simulink model "ADCSSimulator"  (R2024a)
settings: Solver=ode4  StartTime=0.0  StopTime=600  FixedStep=0.01  MaxStep=0.1  RelTol=1e-3  AbsTol=1e-3
values from neighbouring files (symbols this model uses):
  ActuatorAllocationMatrix = ActuatorPhysicalMatrix' * inv(ActuatorPhysicalMatrix * ActuatorPhysicalMatrix')    [set_Init.m]
  ActuatorPhysicalMatrix = [1, 0, 0, 0 ... (first row only)    [set_Init.m]
  albedo_irradiance = 300    [set_Init.m]
  b = 0    [set_Init.m]
  Cd = 2.2    [set_Init.m]
  h_bias = [0; 0; 0]    [set_Init.m]
  J = 4.0e-3 / 628    (= 6.36942675159e-06)    [set_Init.m]
  k_Bdot = ((4 * pi * 0.5236 * 0.0055) / (5677.2 * (4.5e-5)^2))    (= 3147.8423197)    [set_Init.m]
  K_E = K_T    (= 0.0022)    [set_Init.m]
  K_T = 0.0022    [set_Init.m]
  P0 = blkdiag(P0_att, P0_bias)    [set_Init.m]
  P0_att = eye(3) * initial_variance_rad2    [set_Init.m]
  PowerVoltageBus_01 = 3.3    [set_Init.m]
  PowerVoltageBus_02 = 3.3    [set_Init.m]
  PowerVoltageBus_03 = 3.3    [set_Init.m]
  PowerVoltageBus_04 = 3.3    [set_Init.m]
  PowerVoltageBus_05 = 3.3    [set_Init.m]
  PowerVoltageBus_06 = 3.3    [set_Init.m]
  PowerVoltageBus_07 = 3.3    [set_Init.m]
  PowerVoltageBus_08 = 3.3    [set_Init.m]
  PowerVoltageBus_09 = 3.3    [set_Init.m]
  PowerVoltageBus_10 = 3.3    [set_Init.m]
  PowerVoltageBus_11 = 3.3    [set_Init.m]
  PowerVoltageBus_12 = 0.0    (= 0)    [set_Init.m]
  PowerVoltageBus_13 = 0.0    (= 0)    [set_Init.m]
  PowerVoltageBus_14 = 0.0    (= 0)    [set_Init.m]
  PowerVoltageBus_15 = 0.0    (= 0)    [set_Init.m]
  R = 2.0    (= 2)    [set_Init.m]
  ressidual_m = [3e-4; -2e-4; 1e-4]    [set_Init.m]
  solar_irradiance = 1361    [set_Init.m]
  surface_areas = [A_xy, A_yz, A_xz, A_xy, A_yz, A_xz]    [set_Init.m]
  surface_normals_body = [eye(3) -eye(3)]    [set_Init.m]
  surface_positions_body = [       hx,   0,   0 ... (first row only)    [set_Init.m]
  surface_reflectivities = [0.9 0.8 0.9 0.9 0.9 0.9]    [set_Init.m]
  Switch_01 = 1    [set_Init.m]
  Switch_02 = 1    [set_Init.m]
  Switch_03 = 1    [set_Init.m]
  Switch_04 = 1    [set_Init.m]
  Switch_05 = 1    [set_Init.m]
  Switch_06 = 1    [set_Init.m]
  Switch_07 = 1    [set_Init.m]
  Switch_08 = 1    [set_Init.m]
  Switch_09 = 1    [set_Init.m]
  Switch_10 = 1    [set_Init.m]
  Switch_11 = 1    [set_Init.m]
  Switch_12 = 0    [set_Init.m]
  Switch_13 = 0    [set_Init.m]
  Switch_14 = 0    [set_Init.m]
  Switch_15 = 0    [set_Init.m]
  visSampleTime = 0.1    [set_Init.m]
undefined symbols (not defined in the file or in its folder): attitude, Controller, epoch, IAU, juliandate, Kd, km, Kp, m, rad, s, satellite, SGP4_parameters, simulator, UKF_parameters, WMM2020
libraries: sharedtransform x27, aerolibutil x22, aerolibconvert2 x18, simulink_extras x16, matrix_library x6, aerolibtransform2 x4, vrlib x2, aerolibgravity2 x2, aerolibobsolete x1, aerolibattitudesys x1, simulink x1
(part 1 of 8)
settings Model: Creator=dani  LastModifiedBy=dani

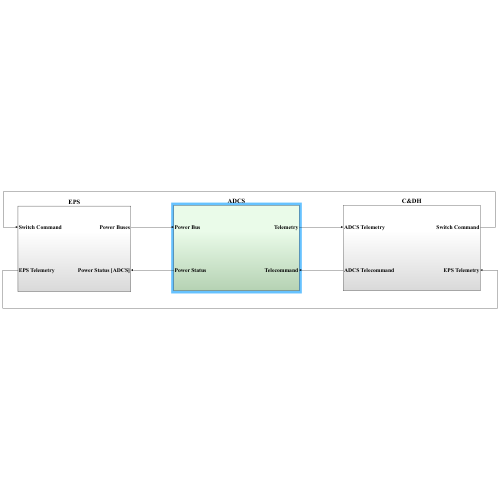
[thumbnail: Simulink's stored preview of the top-level diagram]
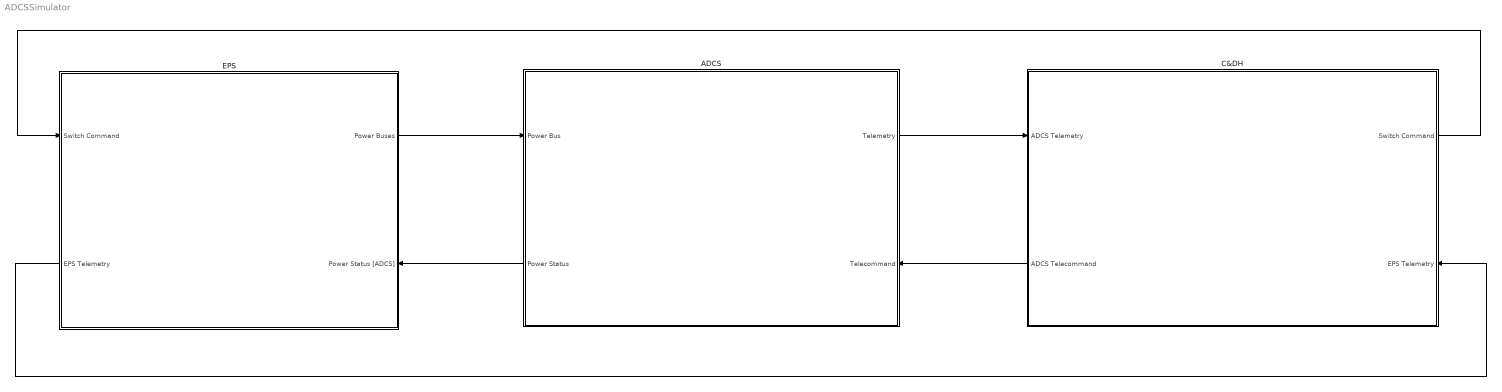
== system ADCSSimulator ==
  ADCS : Subsystem
      settings: PortSchema="{\"entries\":[{\"content\":{\"sides\":[{\"content\":{\"connectorIds\":[\"In1\",\"Out2\"]},\"type\":\"ConnectorPlacement.EquallySpacedRectSide\",\"uuid\":\"aa3848c2-740f-4ead-a432-f3c79fc9daf0\"},{\"content\":{\"connectorIds\":[\"Out1\",\"In2\"],\"side\":\"RIGHT\"},\"type\":\"ConnectorPlacement.EquallySpacedRectSide\",\"uuid\":\"c96c275d-03b5-4d03-9fcd-7be32dac6d00\"},{\"content\":{\"side\":\"TOP\"},\"type\":\"ConnectorPlacement.EquallySpacedRectSide\",\"uuid\":\"31331525-31c2-42c0-b454-d98af43a0c1b\"},{\"content\":{\"side\":\"BOTTOM\"},\"type\":\"ConnectorPlacement.EquallySpacedRectSide\",\"uuid\":\"eb70cc62-5643-48b5-a59b-44e32afdbd5b\"}]},\"type\":\"ConnectorPlacement.EquallySpacedConnector\",\"uuid\":\"a031f488-e476-44b2-bfa5-ca27c87ecf65\"}],\"packageUris\":[\"http://schema.mathworks.com/mf0/Connector/R2020b\"],\"version\":\"1.0\"}"
  C&DH : Subsystem
      settings: PortSchema="{\"entries\":[{\"content\":{\"sides\":[{\"content\":{\"connectorIds\":[\"In1\",\"Out2\"]},\"type\":\"ConnectorPlacement.EquallySpacedRectSide\",\"uuid\":\"3ad3e378-21eb-4eff-b41a-c92f181c1ecc\"},{\"content\":{\"connectorIds\":[\"Out1\",\"In2\"],\"side\":\"RIGHT\"},\"type\":\"ConnectorPlacement.EquallySpacedRectSide\",\"uuid\":\"0538179f-4ab0-45db-a75e-d38723b4a5a1\"},{\"content\":{\"side\":\"TOP\"},\"type\":\"ConnectorPlacement.EquallySpacedRectSide\",\"uuid\":\"084a5a74-d737-4e15-943a-c0ca9c781568\"},{\"content\":{\"side\":\"BOTTOM\"},\"type\":\"ConnectorPlacement.EquallySpacedRectSide\",\"uuid\":\"08c1cc82-b359-4a4d-a3dd-2424cb8433d7\"}]},\"type\":\"ConnectorPlacement.EquallySpacedConnector\",\"uuid\":\"d1795a99-1dc8-4811-af35-3434a23822bd\"}],\"packageUris\":[\"http://schema.mathworks.com/mf0/Connector/R2020b\"],\"version\":\"1.0\"}"
  EPS : Subsystem
      settings: PortSchema="{\"entries\":[{\"content\":{\"sides\":[{\"content\":{\"connectorIds\":[\"In1\",\"Out2\"]},\"type\":\"ConnectorPlacement.EquallySpacedRectSide\",\"uuid\":\"3ad3e378-21eb-4eff-b41a-c92f181c1ecc\"},{\"content\":{\"connectorIds\":[\"Out1\",\"In2\"],\"side\":\"RIGHT\"},\"type\":\"ConnectorPlacement.EquallySpacedRectSide\",\"uuid\":\"0538179f-4ab0-45db-a75e-d38723b4a5a1\"},{\"content\":{\"side\":\"TOP\"},\"type\":\"ConnectorPlacement.EquallySpacedRectSide\",\"uuid\":\"084a5a74-d737-4e15-943a-c0ca9c781568\"},{\"content\":{\"side\":\"BOTTOM\"},\"type\":\"ConnectorPlacement.EquallySpacedRectSide\",\"uuid\":\"08cac11b-dd67-4d0a-9adb-ddefdbada8d1\"}]},\"type\":\"ConnectorPlacement.EquallySpacedConnector\",\"uuid\":\"d1795a99-1dc8-4811-af35-3434a23822bd\"}],\"packageUris\":[\"http://schema.mathworks.com/mf0/Connector/R2020b\"],\"version\":\"1.0\"}"
  wires:
  C&DH/2(ADCS Telecommand) -> ADCS/2(Telecommand)
  ADCS/2(Power Status) -> EPS/2(Power Status [ADCS])
  EPS/1(Power Buses) -> ADCS/1(Power Bus)
  C&DH/1(Switch Command) -> EPS/1(Switch Command)
  ADCS/1(Telemetry) -> C&DH/1(ADCS Telemetry)
  EPS/2(EPS Telemetry) -> C&DH/2(EPS Telemetry)

== system ADCSSimulator/ADCS ==
  note: Temporary Signal
      | (Only for Comparison)
  Power Bus : Inport
  Telecommand : Inport  Port=2
  ADCS Hardware : Subsystem
      settings: PortSchema="{\"entries\":[{\"content\":{\"sides\":[{\"content\":{\"connectorIds\":[\"In1\",\"In2\",\"Out3\"]},\"type\":\"ConnectorPlacement.EquallySpacedRectSide\",\"uuid\":\"766d0d2c-d357-4ba2-aa5f-dc26e66264eb\"},{\"content\":{\"connectorIds\":[\"Out1\",\"Out2\",\"In3\"],\"side\":\"RIGHT\"},\"type\":\"ConnectorPlacement.EquallySpacedRectSide\",\"uuid\":\"3ef54b5b-eb3f-4ad4-b707-91b0a7134d5c\"},{\"content\":{\"side\":\"TOP\"},\"type\":\"ConnectorPlacement.EquallySpacedRectSide\",\"uuid\":\"06ee7821-1a08-4071-958f-cf5282d5f19e\"}]},\"type\":\"ConnectorPlacement.EquallySpacedConnector\",\"uuid\":\"44073966-09cf-4676-b7c4-ea8934a60606\"}],\"packageUris\":[\"http://schema.mathworks.com/mf0/Connector/R2020b\"],\"version\":\"1.0\"}"
  ADCS Software : Subsystem
      settings: PortSchema="{\"entries\":[{\"content\":{\"sides\":[{\"content\":{\"connectorIds\":[\"In1\",\"In2\"]},\"type\":\"ConnectorPlacement.EquallySpacedRectSide\",\"uuid\":\"a2366055-7441-4d66-9a67-a5a05521bed6\"},{\"content\":{\"connectorIds\":[\"Out1\",\"Out2\"],\"side\":\"RIGHT\"},\"type\":\"ConnectorPlacement.EquallySpacedRectSide\",\"uuid\":\"d11468d0-ec53-4005-81d6-c107e48fef08\"},{\"content\":{\"connectorIds\":[\"In3\",\"In4\"],\"side\":\"TOP\"},\"type\":\"ConnectorPlacement.EquallySpacedRectSide\",\"uuid\":\"0424b65d-589c-439a-af82-86bada1149e6\"}]},\"type\":\"ConnectorPlacement.EquallySpacedConnector\",\"uuid\":\"691de30c-3ace-413d-83af-9a4acbe20075\"}],\"packageUris\":[\"http://schema.mathworks.com/mf0/Connector/R2020b\"],\"version\":\"1.0\"}"
  Environment Model : Subsystem
  Telemetry : Outport
  Power Status : Outport  Port=2
  wires:
  Telecommand/1 -> ADCS Software/1(Command)
  Power Bus/1 -> ADCS Hardware/2(Voltage Bus)
  Environment Model/1(Environment) -> ADCS Software/3(Environment), ADCS Hardware/3(True Physical State)
  ADCS Software/1(Actuators Command) -> ADCS Hardware/1(Control Command)
  ADCS Hardware/1(Actuators Command) -> Environment Model/1(Control Torque), ADCS Software/4(Actuators Feedback)
  ADCS Hardware/3(Sensors Data) -> ADCS Software/2(Sensors Data)
  ADCS Software/2(Telemetry) -> Telemetry/1
  ADCS Hardware/2(Power Status) -> Power Status/1

== system ADCSSimulator/C&DH ==
  ADCS Telemetry : Inport
  EPS Telemetry : Inport  Port=2
  Bus Creator : BusCreator  Inputs=15
  Bus Selector : BusSelector  OutputSignals=SOC,Total Instantaneous Power (W),Total Instantaneous Current (A)
  Constant : Constant  Value=Switch_01
  Constant1 : Constant  Value=Switch_02
  Constant10 : Constant  Value=Switch_11
  Constant11 : Constant  Value=Switch_12
  Constant12 : Constant  Value=Switch_13
  Constant13 : Constant  Value=Switch_14
  Constant14 : Constant  Value=Switch_15
  Constant2 : Constant  Value=Switch_03
  Constant3 : Constant  Value=Switch_04
  Constant4 : Constant  Value=Switch_05
  Constant5 : Constant  Value=Switch_06
  Constant6 : Constant  Value=Switch_07
  Constant7 : Constant  Value=Switch_08
  Constant8 : Constant  Value=Switch_09
  Constant9 : Constant  Value=Switch_10
  System Mode (0: OFF) (1: Detumbling) (2: Nadir Pointing) (3: Sun Pointing) : Constant  Value=0
  Terminator : Terminator
  To Workspace : ToWorkspace  VariableName=SOC  SaveFormat=Timeseries  SampleTime=-1
  To Workspace1 : ToWorkspace  VariableName=totoal_p  SaveFormat=Timeseries  SampleTime=-1
  To Workspace2 : ToWorkspace  VariableName=total_I  SaveFormat=Timeseries  SampleTime=-1
  Switch Command : Outport
  ADCS Telecommand : Outport  Port=2
  wires:
  System Mode (0: OFF) (1: Detumbling) (2: Nadir Pointing) (3: Sun Pointing)/1 -> ADCS Telecommand/1
  Constant11/1 -> Bus Creator/12  "Switch 12"
  Constant4/1 -> Bus Creator/5  "Switch 05"
  Constant9/1 -> Bus Creator/10  "Switch 10"
  Constant14/1 -> Bus Creator/15  "Switch 15"
  Constant2/1 -> Bus Creator/3  "Switch 03"
  Constant7/1 -> Bus Creator/8  "Switch 08"
  Constant/1 -> Bus Creator/1  "Switch 01"
  Bus Creator/1 -> Switch Command/1
  Constant12/1 -> Bus Creator/13  "Switch 13"
  Constant3/1 -> Bus Creator/4  "Switch 04"
  Constant1/1 -> Bus Creator/2  "Switch 02"
  Constant5/1 -> Bus Creator/6  "Switch 06"
  Constant6/1 -> Bus Creator/7  "Switch 07"
  Constant13/1 -> Bus Creator/14  "Switch 14"
  Constant10/1 -> Bus Creator/11  "Switch 11"
  Constant8/1 -> Bus Creator/9  "Switch 09"
  ADCS Telemetry/1 -> Terminator/1
  EPS Telemetry/1 -> Bus Selector/1
  Bus Selector/1 -> To Workspace/1  "<SOC>"
  Bus Selector/2 -> To Workspace1/1  "<Total Instantaneous Power (W)>"
  Bus Selector/3 -> To Workspace2/1  "<Total Instantaneous Current (A)>"

== system ADCSSimulator/EPS ==
  Switch Command : Inport
  Power Status [ADCS] : Inport  Port=2
  EPS HouseKeeping : Subsystem
  Power Distribution Unit (PDU) : Subsystem
  Power Buses : Outport
  EPS Telemetry : Outport  Port=2
  wires:
  Switch Command/1 -> [SwitchCommand], Power Distribution Unit (PDU)/1(Switch Bus)
  [SwitchCommand] -> EPS HouseKeeping/1(Switch Status)
  Power Status [ADCS]/1 -> EPS HouseKeeping/2(Power Status)
  EPS HouseKeeping/1(EPS Telemetry) -> EPS Telemetry/1
  Power Distribution Unit (PDU)/1(Voltage Bus) -> Power Buses/1

== system ADCSSimulator/ADCS/ADCS Hardware ==
  Control Command : Inport
  Voltage Bus : Inport  Port=2
  True Physical State : Inport  Port=3
  Actuators : Subsystem
  Bus Creator : BusCreator  Inputs=3
  Bus Selector1 : BusSelector  OutputSignals=MTQs.MTQs Power Status,RWs.RWs Power Status
  Bus Selector2 : BusSelector  OutputSignals=Sensors Power Status
  Bus Selector3 : BusSelector  OutputSignals=|
      | Calendar,Ephemerides.Satellite Ephemeris [ICRF],Satellite Attitude,Eclipse,Magnetic Field (T).MagneticField
      | (T)[Body],Ephemerides.Planetary Ephemeris [ICRF].Sun Ephemeris [ICRF],Transformers
  Bus Selector4 : BusSelector  OutputSignals=MTQs.Dipoles (Am^2),MTQs.MTQs Power Status.Power Consumption [Magnetorquer Z].Current (A),MTQs.MTQs Power Status.Power Consumption [Magnetorquer Y].Current (A),MTQs.MTQs Power Status.Power Consumption [Magnetorquer X].Current (A),RWs.RWs Angular Velocity [Body].RWs Angular Velocity (RPM).RW#1 Motor Angular Velocity (rad/s),RWs.RWs Angular Velocity [Body].RWs Angular Velocity (RPM).RW#2 Motor Angular Velocity (rad/s),RWs.RWs Angular Velocity [Body].RWs Angular Velocity (RPM).RW#3 Motor Angular Velocity (rad/s),RWs.RWs Torque [Body](Nm)
  Constant1 : Constant  Value=satellite.MM.Temperature
  Constant3 : Constant  Value=satellite.Gyro.MeasurementModelDCM
  Constant4 : Constant  Value=satellite.MM.MeasurementModelDCM
  Mux : Mux  Inputs=3
  Mux1 : Mux  Inputs=3
  "Power Bus{2}" : InportShadow  Port=2
  Sensors : Subsystem
  To Workspace : ToWorkspace  VariableName=MTQ_dipoles  SaveFormat=Timeseries  SampleTime=-1
  To Workspace1 : ToWorkspace  VariableName=MTQ_Current  SaveFormat=Timeseries  SampleTime=-1
  To Workspace2 : ToWorkspace  VariableName=RW_angvel  SaveFormat=Timeseries  SampleTime=-1
  To Workspace3 : ToWorkspace  VariableName=RW_Torque  SaveFormat=Timeseries  SampleTime=-1
  Actuators Command : Outport
  Power Status : Outport  Port=2
  Sensors Data : Outport  Port=3
  wires:
  Voltage Bus/1 -> Actuators/2(Input Bus Voltage (V))
  Control Command/1 -> Actuators/1(Control Command)
  Actuators/1(Actuators) -> [Actuators], Actuators Command/1
  [B_Body] -> Actuators/3(Magnetic Field (T))
  Bus Selector2/1 -> Bus Creator/3  "<Sensors Power Status>"
  [Actuators] -> Bus Selector1/1
  [SensorsData] -> Bus Selector2/1
  Bus Selector1/2 -> Bus Creator/2  "<RWs Power Status>"
  Bus Selector1/1 -> Bus Creator/1  "<MTQs Power Status>"
  Bus Creator/1 -> Power Status/1
  Bus Selector3/5 -> [B_Body], Sensors/5(Magnetic Field (T))  "<MagneticField (T)[Body]>"
  Constant4/1 -> Sensors/9(Measurement Model DCM (MM))
  True Physical State/1 -> Bus Selector3/1
  "Power Bus{2}"/1 -> Sensors/11(Input Bus Voltages (V))
  Constant3/1 -> Sensors/10(Measurement Model DCM (Gyro))
  Bus Selector3/3 -> Sensors/3(Satellite Attitude)  "<Satellite Attitude>"
  Bus Selector3/1 -> Sensors/1(Calendar)  "<Calendar>"
  Constant1/1 -> Sensors/8(MM Temperature)
  Sensors/1(Sensrors Out) -> [SensorsData], Sensors Data/1
  Bus Selector3/6 -> Sensors/6(Sun Ephemeris [ICRF])  "<Sun Ephemeris [ICRF]>"
  Bus Selector3/7 -> Sensors/7(Transformers)  "<Transformers>"
  Bus Selector3/2 -> Sensors/2(Satellite Ephemeris)  "<Satellite Ephemeris [ICRF]>"
  Bus Selector3/4 -> Sensors/4(Eclipse)  "<Eclipse>"
  [Actuators] -> Bus Selector4/1
  Bus Selector4/2 -> Mux/1  "<Current (A)>"
  Bus Selector4/1 -> To Workspace/1  "<Dipoles (Am^2)>"
  Bus Selector4/3 -> Mux/2  "<Current (A)>"
  Bus Selector4/4 -> Mux/3  "<Current (A)>"
  Bus Selector4/6 -> Mux1/2  "<RW#2 Motor Angular Velocity (rad/s)>"
  Bus Selector4/5 -> Mux1/1  "<RW#1 Motor Angular Velocity (rad/s)>"
  Bus Selector4/7 -> Mux1/3  "<RW#3 Motor Angular Velocity (rad/s)>"
  Mux/1 -> To Workspace1/1
  Mux1/1 -> To Workspace2/1
  Bus Selector4/8 -> To Workspace3/1  "<RWs Torque [Body](Nm)>"

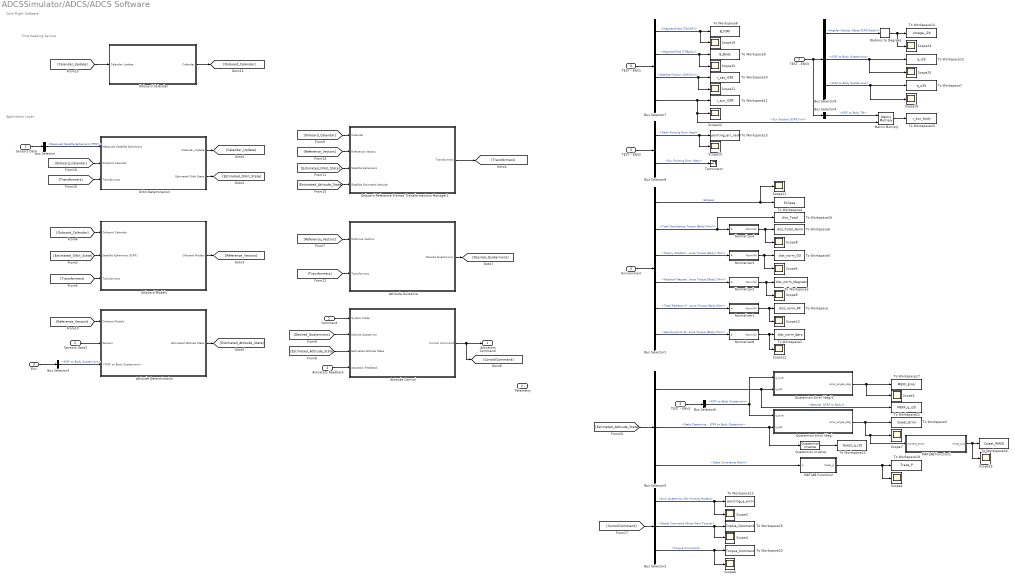
== system ADCSSimulator/ADCS/ADCS Software ==
  note: Time Keeping Service
  note: Core Flight Software
  note: Application Layer
  Command : Inport
  Sensors Data : Inport  Port=2
  Environment : Inport  Port=3
  Actuators Feedback : Inport  Port=4
  Attitude Control : Subsystem
  Attitude Determination : Subsystem
  Attitude Guidance : Subsystem
  Bus Selector : BusSelector  OutputSignals=Measured Satellite Ephemeris [ITRF]
  Bus Selector1 : BusSelector  OutputSignals=Eclipse,Disturbances.Total Disturbance Torque [Body] (Nm),Disturbances.Graciry Gradient Disturbance Torque [Body] (Nm),Disturbances.Residual Magnetic Disturbance Torque [Body] (Nm),Disturbances.Rediation Pressure Torque [Body] (Nm).Total Rediation Pressure Torque [Body](Nm),Disturbances.Aerodynamics Disturbance Torque [Body] (Nm)
  Bus Selector2 : BusSelector  OutputSignals=Error Quaternion [for Pointing Modes],Dipole Command (Given from Torque),Torque Command
  Bus Selector3 : BusSelector  OutputSignals=Transformers.Quaternions.ICRF to Body Quaternions
  Bus Selector4 : BusSelector  OutputSignals=Transformers.Transfer Matrices.ICRF to Body TM
  Bus Selector5 : BusSelector  OutputSignals="Attitude  [ICRF to Body],Static Determination (QUEST): ICRF to Body Quaternion,State Covariance Matrix"
  Bus Selector6 : BusSelector  OutputSignals=Transformers.Quaternions.ICRF to Body Quaternions
  Bus Selector7 : BusSelector  OutputSignals=|
      | Magnetic Field (T).MagneticField
      | (T)[ICRF],Magnetic Field (T).MagneticField
      | (T)[Body],Ephemerides.Satellite Ephemeris [ICRF].Satellite Position [ICRF](m),Ephemerides.Planetary Ephemeris [ICRF].Sun Ephemeris [ICRF].Sun Position [ICRF] (m)
  Bus Selector8 : BusSelector  OutputSignals=Transformers.Pinting Error (Deg).Nadir Pointing Error (deg),Transformers.Pinting Error (Deg).Sun Pointing Error (deg)
  Bus Selector9 : BusSelector  OutputSignals=Satellite Attitude.Angular Velocity {Body-ICRF}(rad/s),Transformers.Quaternions.ICRF to Body Quaternions,Transformers.Quaternions.Orbit to Body Quaternions
  Env : InportShadow  Port=3
  MATLAB Function1 : MATLAB Function  TreatAsAtomicUnit=on  SystemSampleTime=0.1
  MATLAB Function2 : MATLAB Function  TreatAsAtomicUnit=on
  Matrix Multiply : Product  Multiplication=Matrix(*)
  Normalizer1 : Subsystem
  Normalizer2 : Subsystem
  Normalizer3 : Subsystem
  Normalizer4 : Subsystem
  Normalizer8 : Subsystem
  Onboard Calendar : Subsystem
  Onboard Models : Subsystem
  Onboard Reference Frames Transformations Manager1 : Subsystem
  Orbit Detemination : Subsystem
  Quaternion Inverse : aerolibutil/Quaternion Inverse
  Quaternion Error (deg) : MATLAB Function  TreatAsAtomicUnit=on
  Quaternion Error (deg)1 : MATLAB Function  TreatAsAtomicUnit=on
  Radians to Degrees : simulink_extras/Transformations/Radians to Degrees
  Scope{1..12,15,19..26} (21 alike) : Scope
  Sensors Data2 : InportShadow  Port=2
  TEST - ENV{1..4} (4 alike) : InportShadow  Port=3
  Terminator : Terminator
  To Workspace : ToWorkspace  VariableName=dist_norm_RP  SaveFormat=Timeseries  SampleTime=-1
  To Workspace1 : ToWorkspace  VariableName=dist_norm_Aero  SaveFormat=Timeseries  SampleTime=-1
  To Workspace10 : ToWorkspace  VariableName=r_sat_ICRF  SaveFormat=Timeseries  SampleTime=-1
  To Workspace11 : ToWorkspace  VariableName=r_sun_ICRF  SaveFormat=Timeseries  SampleTime=-1
  To Workspace12 : ToWorkspace  VariableName=pointing_q_error  SaveFormat=Timeseries  SampleTime=-1
  To Workspace13 : ToWorkspace  VariableName=pointing_err_nadir  SaveFormat=Timeseries  SampleTime=-1
  To Workspace14 : ToWorkspace  VariableName=omega_i2b  SaveFormat=Timeseries  SampleTime=-1
  To Workspace15 : ToWorkspace  VariableName=q_i2b  SaveFormat=Timeseries  SampleTime=-1
  To Workspace16 : ToWorkspace  VariableName=dist_Total  SaveFormat=Timeseries  SampleTime=-1
  To Workspace17 : ToWorkspace  VariableName=MEKF_Error  SaveFormat=Timeseries  SampleTime=-1
  To Workspace18 : ToWorkspace  VariableName=Trace_P  SaveFormat=Timeseries  SampleTime=-1
  To Workspace19 : ToWorkspace  VariableName=Dipole_Command  SaveFormat=Timeseries  SampleTime=-1
  To Workspace2 : ToWorkspace  VariableName=dist_norm_Magnetic  SaveFormat=Timeseries  SampleTime=-1
  To Workspace20 : ToWorkspace  VariableName=Torque_Command  SaveFormat=Timeseries  SampleTime=-1
  To Workspace21 : ToWorkspace  VariableName=MEKF_q_i2b  SaveFormat=Timeseries  SampleTime=-1
  To Workspace22 : ToWorkspace  VariableName=Quest_q_i2b  SaveFormat=Timeseries  SampleTime=-1
  To Workspace23 : ToWorkspace  VariableName=r_sun_body  SaveFormat=Timeseries  SampleTime=-1
  To Workspace24 : ToWorkspace  VariableName=Quest_RMSE  SaveFormat=Timeseries  SampleTime=-1
  To Workspace3 : ToWorkspace  VariableName=Quest_Error  SaveFormat=Timeseries  SampleTime=-1
  To Workspace4 : ToWorkspace  VariableName=Eclipse  SaveFormat=Timeseries  SampleTime=-1
  To Workspace5 : ToWorkspace  VariableName=dist_norm_GG  SaveFormat=Timeseries  SampleTime=-1
  To Workspace6 : ToWorkspace  VariableName=dist_Total_Norm  SaveFormat=Timeseries  SampleTime=-1
  To Workspace7 : ToWorkspace  VariableName=q_o2b  SaveFormat=Timeseries  SampleTime=-1
  To Workspace8 : ToWorkspace  VariableName=B_ICRF  SaveFormat=Timeseries  SampleTime=-1
  To Workspace9 : ToWorkspace  VariableName=B_Body  SaveFormat=Timeseries  SampleTime=-1
  Actuators Command : Outport
  Telemetry : Outport  Port=2
  wires:
  [Calendar_Update] -> Onboard Calendar/1(Calendar Update)
  Onboard Calendar/1(Calendar) -> [Onboard_Calendar]
  [Transformers] -> Attitude Guidance/2(Transformers)
  Orbit Detemination/1(Calendar_Update) -> [Calendar_Update]
  [Transformers] -> Onboard Models/3(Transformers)
  [Estimated_Orbit_State] -> Onboard Reference Frames Transformations Manager1/3(Satellite Ephemeris)
  Onboard Reference Frames Transformations Manager1/1(Transformers) -> [Transformers]
  [Onboard_Calendar] -> Onboard Reference Frames Transformations Manager1/1(Calendar)
  [Reference_Vectors] -> Onboard Reference Frames Transformations Manager1/2(Reference Vectors)
  [Reference_Vectors] -> Attitude Determination/1(Onboard Models)
  Sensors Data/1 -> Bus Selector/1
  [Estimated_Attitude_State] -> Onboard Reference Frames Transformations Manager1/4(Satellite Estimated Attitude)
  Command/1 -> Attitude Control/1(System Mode)
  [Estimated_Attitude_State] -> Attitude Control/3(Estimated Attitude State)
  Attitude Determination/1(Estimated Attitude State) -> [Estimated_Attitude_State]
  Attitude Guidance/1(Desired Quaternions) -> [Desired_Quaternions]
  Onboard Models/1(Onboard Models) -> [Reference_Vectors]
  Bus Selector/1 -> Orbit Detemination/1(Measured Satellite Ephemeris)  "<Measured Satellite Ephemeris [ITRF]>"
  [Onboard_Calendar] -> Onboard Models/1(Onboard Calendar)
  Attitude Control/1(Control Command) -> [ControlCommand], Actuators Command/1
  Orbit Detemination/2(Estimated Orbit State) -> [Estimated_Orbit_State]
  [Desired_Quaternions] -> Attitude Control/2(Desired Quaternion)
  Sensors Data2/1 -> Attitude Determination/2(Sensors)
  [Reference_Vectors] -> Attitude Guidance/1(Refernce Vectors)
  [Transformers] -> Orbit Detemination/3(Transformers)
  [Onboard_Calendar] -> Orbit Detemination/2(Onboard Calendar)
  [Estimated_Orbit_State] -> Onboard Models/2(Satellite Ephemeris [ICRF])
  [Estimated_Attitude_State] -> Bus Selector5/1
  Bus Selector5/1 -> To Workspace21/1, Quaternion Error (deg)1/2(q_est)  "<Attitude  [ICRF to Body]>"
  Bus Selector6/1 -> Quaternion Error (deg)1/1(q_true), Quaternion Error (deg)/1(q_true)  "<ICRF to Body Quaternions>"
  Quaternion Error (deg)/1(error_angle_deg) -> MATLAB Function1/1(current_error), Scope7/1, To Workspace3/1
  Environment/1 -> Bus Selector1/1
  Bus Selector1/1 -> Scope11/1, To Workspace4/1  "<Eclipse>"
  Bus Selector5/2 -> Quaternion Inverse/1, Quaternion Error (deg)/2(q_est)  "<Static Determination (QUEST): ICRF to Body Quaternion>"
  Bus Selector1/2 -> To Workspace16/1, Normalizer4/1(A)  "<Total Disturbance Torque [Body] (Nm)>"
  Bus Selector1/3 -> Normalizer3/1(A)  "<Graciry Gradient Disturbance Torque [Body] (Nm)>"
  Bus Selector1/4 -> Normalizer2/1(A)  "<Residual Magnetic Disturbance Torque [Body] (Nm)>"
  Bus Selector1/5 -> Normalizer1/1(A)  "<Total Rediation Pressure Torque [Body](Nm)>"
  Bus Selector2/1 -> To Workspace12/1, Scope3/1  "<Error Quaternion [for Pointing Modes]>"
  Bus Selector1/6 -> Normalizer8/1(A)  "<Aerodynamics Disturbance Torque [Body] (Nm)>"
  Normalizer3/1(Norm(A)) -> Scope5/1, To Workspace5/1
  Normalizer2/1(Norm(A)) -> Scope9/1, To Workspace2/1
  Normalizer1/1(Norm(A)) -> Scope10/1, To Workspace/1
  Normalizer8/1(Norm(A)) -> Scope12/1, To Workspace1/1
  Normalizer4/1(Norm(A)) -> To Workspace6/1, Scope8/1
  Bus Selector7/4 -> Matrix Multiply/2, Scope22/1, To Workspace11/1  "<Sun Position [ICRF] (m)>"
  Bus Selector7/3 -> Scope21/1, To Workspace10/1  "<Satellite Position [ICRF](m)>"
  Bus Selector7/2 -> Scope20/1, To Workspace9/1  "<MagneticField (T)[Body]>"
  Bus Selector7/1 -> Scope19/1, To Workspace8/1  "<MagneticField (T)[ICRF]>"
  Bus Selector8/1 -> Scope23/1, To Workspace13/1  "<Nadir Pointing Error (deg)>"
  Bus Selector8/2 -> Terminator/1  "<Sun Pointing Error (deg)>"
  TEST - ENV1/1 -> Bus Selector7/1
  TEST - ENV2/1 -> Bus Selector8/1
  Bus Selector9/2 -> Scope25/1, To Workspace15/1  "<ICRF to Body Quaternions>"
  TEST - ENV3/1 -> Bus Selector4/1, Bus Selector9/1
  Bus Selector9/1 -> Radians to Degrees/1  "<Angular Velocity {Body-ICRF}(rad/s)>"
  Bus Selector9/3 -> Scope26/1, To Workspace7/1  "<Orbit to Body Quaternions>"
  Radians to Degrees/1 -> Scope24/1, To Workspace14/1
  TEST - ENV4/1 -> Bus Selector6/1
  Env/1 -> Bus Selector3/1
  Bus Selector3/1 -> Attitude Determination/3(<ICRF to Body Quaternions>)  "<ICRF to Body Quaternions>"
  Quaternion Error (deg)1/1(error_angle_deg) -> Scope1/1, To Workspace17/1
  Bus Selector5/3 -> MATLAB Function2/1(p)  "<State Covariance Matrix>"
  MATLAB Function2/1(trace_p) -> Scope2/1, To Workspace18/1
  [ControlCommand] -> Bus Selector2/1
  Bus Selector2/2 -> To Workspace19/1, Scope4/1  "<Dipole Command (Given from Torque)>"
  Bus Selector2/3 -> Scope6/1, To Workspace20/1  "<Torque Command>"
  Matrix Multiply/1 -> To Workspace23/1
  Bus Selector4/1 -> Matrix Multiply/1  "<ICRF to Body TM>"
  MATLAB Function1/1(rmse_out) -> Scope15/1, To Workspace24/1
  Quaternion Inverse/1 -> To Workspace22/1
  Actuators Feedback/1 -> Attitude Control/4(Actuators Feedback)

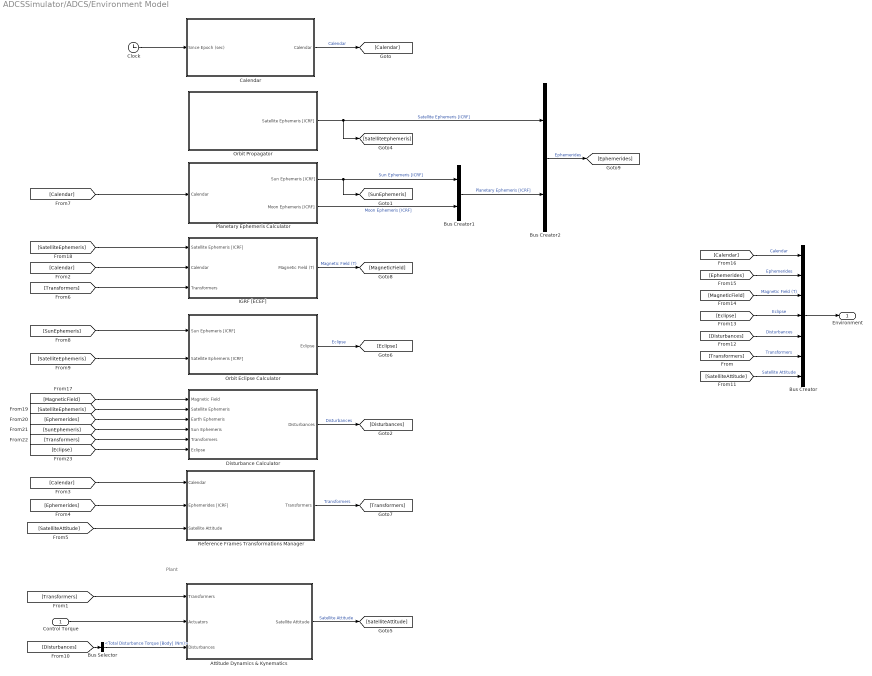
== system ADCSSimulator/ADCS/Environment Model ==
  note: Plant
  Control Torque : Inport
  Attitude Dynamics & Kynematics : Subsystem
  Bus Creator : BusCreator  Inputs=7
  Bus Creator1 : BusCreator  Inputs=2
  Bus Creator2 : BusCreator  Inputs=2
  Bus Selector : BusSelector  OutputSignals=Total Disturbance Torque [Body] (Nm)
  "Calendar " : Subsystem
  Clock : Clock
  Disturbance Calculator : Subsystem
  IGRF [ECEF] : Subsystem
  Orbit Eclipse Calculator : Subsystem
  Orbit Propagator : Subsystem
  Planetary Ephemeris Calculator : Subsystem
  Reference Frames Transformations Manager : Subsystem
  Environment : Outport
  wires:
  [SatelliteEphemeris] -> IGRF [ECEF]/1(Satellite Ephemeris [ICRF])
  Orbit Propagator/1(Satellite Ephemeris [ICRF]) -> [SatelliteEphemeris], Bus Creator2/1  "Satellite Ephemeris [ICRF]"
  Clock/1 -> "Calendar "/1(Since Epoch (sec))
  IGRF [ECEF]/1(Magnetic Field (T)) -> [MagneticField]  "Magnetic Field (T)"
  [Calendar] -> Planetary Ephemeris Calculator/1(Calendar)
  [SunEphemeris] -> Orbit Eclipse Calculator/1(Sun Ephemeris [ICRF])
  [SatelliteEphemeris] -> Orbit Eclipse Calculator/2(Satellite Ephemeris [ICRF])
  Orbit Eclipse Calculator/1(Eclipse) -> [Eclipse]  "Eclipse"
  Bus Creator2/1 -> [Ephemerides]  "Ephemerides"
  "Calendar "/1(Calendar) -> [Calendar]  "Calendar"
  [Calendar] -> IGRF [ECEF]/2(Calendar)
  [Transformers] -> IGRF [ECEF]/3(Transformers)
  Planetary Ephemeris Calculator/1(Sun Ephemeris [ICRF]) -> [SunEphemeris], Bus Creator1/1  "Sun Ephemeris [ICRF]"
  Planetary Ephemeris Calculator/2(Moon Ephemeris [ICRF]) -> Bus Creator1/2  "Moon Ephemeris [ICRF]"
  [Disturbances] -> Bus Selector/1
  [Transformers] -> Attitude Dynamics & Kynematics/1(Transformers)
  Attitude Dynamics & Kynematics/1(Satellite Attitude) -> [SatelliteAttitude]  "Satellite Attitude"
  [Ephemerides] -> Reference Frames Transformations Manager/2(Ephemerides [ICRF])
  [SatelliteAttitude] -> Reference Frames Transformations Manager/3(Satellite Attitude)
  [Calendar] -> Reference Frames Transformations Manager/1(Calendar)
  Reference Frames Transformations Manager/1(Transformers) -> [Transformers]  "Transformers"
  Bus Creator1/1 -> Bus Creator2/2  "Planetary Ephemeris [ICRF]"
  Disturbance Calculator/1(Disturbances) -> [Disturbances]  "Disturbances"
  Control Torque/1 -> Attitude Dynamics & Kynematics/2(Actuators)
  Bus Creator/1 -> Environment/1
  [Transformers] -> Bus Creator/6  "Transformers"
  [SatelliteAttitude] -> Bus Creator/7  "Satellite Attitude"
  [Disturbances] -> Bus Creator/5  "Disturbances"
  [Eclipse] -> Bus Creator/4  "Eclipse"
  [MagneticField] -> Bus Creator/3  "Magnetic Field (T)"
  [Ephemerides] -> Bus Creator/2  "Ephemerides"
  [Calendar] -> Bus Creator/1  "Calendar"
  [Transformers] -> Disturbance Calculator/5(Transformers)
  [SunEphemeris] -> Disturbance Calculator/4(Sun Ephemeris)
  [Ephemerides] -> Disturbance Calculator/3(Earth Ephemeris)
  [SatelliteEphemeris] -> Disturbance Calculator/2(Satellite Ephemeris)
  [MagneticField] -> Disturbance Calculator/1(Magnetic Field)
  Bus Selector/1 -> Attitude Dynamics & Kynematics/3(Disturbances)  "<Total Disturbance Torque [Body] (Nm)>"
  [Eclipse] -> Disturbance Calculator/6(Eclipse)

== system ADCSSimulator/EPS/EPS HouseKeeping ==
  Switch Status : Inport
  Power Status : Inport  Port=2
  Battery : Subsystem
  Bus Creator2 : BusCreator  Inputs=7
  Bus Selector : BusSelector  OutputSignals=MTQs Power Status,RWs Power Status,Sensors Power Status
  Power Telemetry1 : InportShadow  Port=2
  SOC Calculator : Subsystem
      settings: PortSchema="{\"entries\":[{\"content\":{\"sides\":[{\"content\":{\"connectorIds\":[\"In1\"]},\"type\":\"ConnectorPlacement.EquallySpacedRectSide\",\"uuid\":\"f7bc3b4c-451d-493e-8998-a343d0a5a0b2\"},{\"content\":{\"connectorIds\":[\"Out1\"],\"side\":\"RIGHT\"},\"type\":\"ConnectorPlacement.EquallySpacedRectSide\",\"uuid\":\"28b30868-d4a6-47ce-af54-62c45a7f04f8\"},{\"content\":{\"connectorIds\":[\"In2\"],\"side\":\"TOP\"},\"type\":\"ConnectorPlacement.EquallySpacedRectSide\",\"uuid\":\"92fa9cff-9026-4330-960b-573908f25428\"}]},\"type\":\"ConnectorPlacement.EquallySpacedConnector\",\"uuid\":\"b68e6826-a1f7-4c62-98ea-304744d8172e\"}],\"packageUris\":[\"http://schema.mathworks.com/mf0/Connector/R2020b\"],\"version\":\"1.0\"}"
  Total Current Consumption (A) : Subsystem
  Total Instantaneous Power Consumption (W) : Subsystem
  EPS Telemetry : Outport
  wires:
  Total Instantaneous Power Consumption (W)/1(Total Power Consumption (W)) -> [TotalPowerConsumption]
  Power Status/1 -> Total Instantaneous Power Consumption (W)/1(Power Telemetry), Total Current Consumption (A)/1(Power Telemetry)
  [SOC] -> Bus Creator2/2  "SOC"
  [TotalPowerConsumption] -> Bus Creator2/3  "Total Instantaneous Power (W)"
  Total Current Consumption (A)/1(Total Current (A)) -> SOC Calculator/1(Total Current (A)), [TotalCurrentConsumption]
  Bus Selector/2 -> Bus Creator2/6  "<RWs Power Status>"
  Battery/1(Battery capacity) -> SOC Calculator/2(Battery capacity)
  SOC Calculator/1(SOC) -> [SOC]
  Bus Selector/1 -> Bus Creator2/5  "<MTQs Power Status>"
  [TotalCurrentConsumption] -> Bus Creator2/4  "Total Instantaneous Current (A)"
  Switch Status/1 -> Bus Creator2/1  "Switch Status"
  Bus Selector/3 -> Bus Creator2/7  "<Sensors Power Status>"
  Bus Creator2/1 -> EPS Telemetry/1  "EPS HK"
  Power Telemetry1/1 -> Bus Selector/1

== system ADCSSimulator/EPS/Power Distribution Unit (PDU) ==
  Switch Bus : Inport
  Bus Creator : BusCreator  Inputs=15
  Bus Selector3 : BusSelector  OutputSignals=Switch 01,Switch 02,Switch 03,Switch 04,Switch 05,Switch 06,Switch 07,Switch 08,Switch 09,Switch 10,Switch 11,Switch 12,Switch 13,Switch 14,Switch 15
  Constraint : Constant  Value=0
  Power Bus #1 : Constant  Value=PowerVoltageBus_01
  Power Bus #10 : Constant  Value=PowerVoltageBus_10
  Power Bus #11 : Constant  Value=PowerVoltageBus_11
  Power Bus #12 : Constant  Value=PowerVoltageBus_12
  Power Bus #13 : Constant  Value=PowerVoltageBus_13
  Power Bus #14 : Constant  Value=PowerVoltageBus_14
  Power Bus #15 : Constant  Value=PowerVoltageBus_15
  Power Bus #2 : Constant  Value=PowerVoltageBus_02
  Power Bus #3 : Constant  Value=PowerVoltageBus_03
  Power Bus #4 : Constant  Value=PowerVoltageBus_04
  Power Bus #5 : Constant  Value=PowerVoltageBus_05
  Power Bus #6 : Constant  Value=PowerVoltageBus_06
  Power Bus #7 : Constant  Value=PowerVoltageBus_07
  Power Bus #8 : Constant  Value=PowerVoltageBus_08
  Power Bus #9 : Constant  Value=PowerVoltageBus_09
  Switch{,1..14} (15 alike) : Switch  Criteria=u2 > Threshold  SaturateOnIntegerOverflow=off  InputSameDT=off
  Voltage Bus : Outport
  wires:
  Switch/1 -> Bus Creator/1  "Power Bus: Sun Sensors"
  Bus Selector3/15 -> Switch14/2  "<Switch 15>"
  Constraint/1 -> Switch14/3, Switch10/3, Switch4/3, Switch3/3, Switch1/3, Switch/3, Switch2/3, Switch5/3, Switch6/3, Switch7/3, Switch8/3, Switch9/3, Switch11/3, Switch12/3, Switch13/3
  Power Bus #1/1 -> Switch/1
  Bus Selector3/4 -> Switch3/2  "<Switch 04>"
  Power Bus #6/1 -> Switch5/1
  Switch3/1 -> Bus Creator/4  "Power Bus: GNSS"
  Bus Selector3/1 -> Switch/2  "<Switch 01>"
  Power Bus #2/1 -> Switch1/1
  Bus Selector3/6 -> Switch5/2  "<Switch 06>"
  Switch2/1 -> Bus Creator/3  "Power Bus: Gyrospcopes"
  Power Bus #5/1 -> Switch4/1
  Bus Selector3/2 -> Switch1/2  "<Switch 02>"
  Switch6/1 -> Bus Creator/7  "Power Bus: RW#3"
  Power Bus #8/1 -> Switch7/1
  Bus Selector3/9 -> Switch8/2  "<Switch 09>"
  Switch5/1 -> Bus Creator/6  "Power Bus: RW#2"
  Switch1/1 -> Bus Creator/2  "Power Bus: Magnetometers"
  Bus Selector3/8 -> Switch7/2  "<Switch 08>"
  Bus Selector3/3 -> Switch2/2  "<Switch 03>"
  Power Bus #4/1 -> Switch3/1
  Switch10/1 -> Bus Creator/11  "Power Bus: MTQ_Z"
  Switch7/1 -> Bus Creator/8  "Power Bus: RW#4"
  Switch8/1 -> Bus Creator/9  "Power Bus: MTQ_X"
  Bus Selector3/5 -> Switch4/2  "<Switch 05>"
  Power Bus #3/1 -> Switch2/1
  Power Bus #9/1 -> Switch8/1
  Bus Selector3/13 -> Switch12/2  "<Switch 13>"
  Switch9/1 -> Bus Creator/10  "Power Bus: MTQ_Y"
  Power Bus #7/1 -> Switch6/1
  Switch12/1 -> Bus Creator/13  "Power Bus: {NOT ALLOCATED}"
  Bus Selector3/12 -> Switch11/2  "<Switch 12>"
  Switch13/1 -> Bus Creator/14  "Power Bus: {NOT ALLOCATED}"
  Switch11/1 -> Bus Creator/12  "Power Bus: {NOT ALLOCATED}"
  Power Bus #10/1 -> Switch9/1
  Power Bus #15/1 -> Switch14/1
  Bus Selector3/7 -> Switch6/2  "<Switch 07>"
  Switch14/1 -> Bus Creator/15  "Power Bus: {NOT ALLOCATED}"
  Switch4/1 -> Bus Creator/5  "Power Bus: RW#1"
  Power Bus #11/1 -> Switch10/1
  Power Bus #13/1 -> Switch12/1
  Power Bus #12/1 -> Switch11/1
  Bus Selector3/10 -> Switch9/2  "<Switch 10>"
  Bus Selector3/14 -> Switch13/2  "<Switch 14>"
  Power Bus #14/1 -> Switch13/1
  Bus Selector3/11 -> Switch10/2  "<Switch 11>"
  Switch Bus/1 -> Bus Selector3/1
  Bus Creator/1 -> Voltage Bus/1  "Voltage Bus"

== system ADCSSimulator/ADCS/ADCS Hardware/Actuators ==
  Control Command : Inport
  Input Bus Voltage (V) : Inport  Port=2
  Magnetic Field (T) : Inport  Port=3
  Bus Creator : BusCreator  Inputs=2
  Bus Selector : BusSelector  OutputSignals=Dipole Command (Given from Torque),Torque Command
  "Power Bus{2}" : InportShadow  Port=2
  Reaction Wheels Model (RWs) : Subsystem
  Tri-axial Magnetorquer Model (MTQs) : Subsystem
  Actuators : Outport
  wires:
  Tri-axial Magnetorquer Model (MTQs)/1(Acutators: MTQs) -> Bus Creator/1  "MTQs"
  Reaction Wheels Model (RWs)/1(Acutators: RWs) -> Bus Creator/2  "RWs"
  Bus Creator/1 -> Actuators/1
  Magnetic Field (T)/1 -> Tri-axial Magnetorquer Model (MTQs)/1(Magnetic Field [Body] (T))
  Input Bus Voltage (V)/1 -> Tri-axial Magnetorquer Model (MTQs)/3(Bus Voltage)
  Bus Selector/1 -> Tri-axial Magnetorquer Model (MTQs)/2(MTQ CMD (A.m^2))  "<Dipole Command (Given from Torque)>"
  "Power Bus{2}"/1 -> Reaction Wheels Model (RWs)/1(RWs Bus Voltage (V))
  Bus Selector/2 -> Reaction Wheels Model (RWs)/2(RWs CMD [Body](N.m))  "<Torque Command>"
  Control Command/1 -> Bus Selector/1

== system ADCSSimulator/ADCS/ADCS Hardware/Sensors ==
  Calendar : Inport
  Satellite Ephemeris : Inport  Port=2
  Satellite Attitude : Inport  Port=3
  Eclipse : Inport  Port=4
  Magnetic Field (T) : Inport  Port=5
  Sun Ephemeris [ICRF] : Inport  Port=6
  Transformers : Inport  Port=7
  MM Temperature : Inport  Port=8
  Measurement Model DCM (MM) : Inport  Port=9
  Measurement Model DCM (Gyro) : Inport  Port=10
  Input Bus Voltages (V) : Inport  Port=11
  Analog Magnetometer Model : Subsystem  Commented=on
  Bus Creator : BusCreator  Inputs=4
  Bus Creator1 : BusCreator  Inputs=5
  Bus Selector : BusSelector  OutputSignals=Angular Velocity {Body-ICRF}(rad/s)
  Bus Selector1 : BusSelector  OutputSignals=Sun Position [ICRF] (m)
  Bus Selector2 : BusSelector  OutputSignals=Quaternions.ICRF to Body Quaternions
  Bus Selector3 : BusSelector  OutputSignals=Transfer Matrices.ICRF to ITRF TM
  Bus Selector4 : BusSelector  OutputSignals=Power Bus: Sun Sensors (signal 1)
  Bus Selector5 : BusSelector  OutputSignals=Power Bus: Magnetometers (signal 2)
  Bus Selector6 : BusSelector  OutputSignals=Power Bus: Gyrospcopes (signal 3)
  Bus Selector7 : BusSelector  OutputSignals=Power Bus: GNSS (signal 4)
  Digital Magnetometer Model : Subsystem
  GNSS Receiver Model : Subsystem
  Gyroscope Model : Subsystem
  Sun Sensor Model : Subsystem  TreatAsAtomicUnit=on
  Transformers1 : InportShadow  Port=7
  Sensrors Out : Outport
  wires:
  Bus Creator/1 -> Bus Creator1/5  "Sensors Power Status"
  [InputVoltage] -> Bus Selector4/1
  [InputVoltage] -> Bus Selector7/1
  Bus Selector2/1 -> Sun Sensor Model/2(q [ICRF to Body])  "<ICRF to Body Quaternions>"
  [PC_Gyroscope] -> Bus Creator/1  "Power Consumption [Gyroscope]"
  [PC_GPS] -> Bus Creator/2  "Power Consumption [GNSS Receiver]"
  Magnetic Field (T)/1 -> Digital Magnetometer Model/1(Magnetic Field [Body] (T))  "real"
  [PC_SunSensor] -> Bus Creator/4  "Power Consumption [Sun Sensor]"
  Satellite Ephemeris/1 -> GNSS Receiver Model/3(Satellite Ephemeris)
  Measurement Model DCM (Gyro)/1 -> Gyroscope Model/3(Measurement Model DCM)
  Input Bus Voltages (V)/1 -> [InputVoltage], Bus Selector5/1
  Sun Sensor Model/2(Power Consumption) -> [PC_SunSensor]  "Power Consumption [Sun Sensor]"
  Sun Sensor Model/1(Measured Sun Vector [Body] (m)) -> Bus Creator1/1  "Measured Sun Vector [Body] (m)"
  [InputVoltage] -> Bus Selector6/1
  Bus Creator1/1 -> Sensrors Out/1
  Gyroscope Model/1(Measured Angular Velocity [Body] (rad/s)) -> Bus Creator1/3  "Measured Angular Velocity [Body] (rad/s)"
  Digital Magnetometer Model/1(Measured Magnetic Field [Body] (T)) -> Bus Creator1/2  "Measured Magnetic Field [Body] (T)"
  Satellite Attitude/1 -> Bus Selector/1
  Bus Selector/1 -> Gyroscope Model/1(Angular Velocity [Body] (rad/s))  "<Angular Velocity {Body-ICRF}(rad/s)>"
  GNSS Receiver Model/2(Power Consumption) -> [PC_GPS]  "Power Consumption [GNSS Receiver]"
  [PC_Magnetometer] -> Bus Creator/3  "Power Consumption [Magnetometer]"
  Transformers/1 -> Bus Selector2/1
  Sun Ephemeris [ICRF]/1 -> Bus Selector1/1
  GNSS Receiver Model/1(Measured Satellite Ephemeris) -> Bus Creator1/4  "Measured Satellite Ephemeris [ITRF]"
  Bus Selector1/1 -> Sun Sensor Model/3(Sun Position [ICRF] (m))  "<Sun Position [ICRF] (m)>"
  Eclipse/1 -> Sun Sensor Model/1(Eclipse)
  Calendar/1 -> GNSS Receiver Model/1(Calendar)
  Gyroscope Model/2(Power Consumption) -> [PC_Gyroscope]  "Power Consumption [Gyroscope]"
  Digital Magnetometer Model/2(Power Consumption) -> [PC_Magnetometer]  "Power Consumption [Magnetometer]"
  Measurement Model DCM (MM)/1 -> Digital Magnetometer Model/4(Measurement Model DCM)
  MM Temperature/1 -> Digital Magnetometer Model/2(Temperature (˚C))
  Bus Selector5/1 -> Digital Magnetometer Model/3(Input Voltage (V))  "<Power Bus: Magnetometers (signal 2)>"
  Bus Selector4/1 -> Sun Sensor Model/4(Input Voltage (V))  "<Power Bus: Sun Sensors (signal 1)>"
  Bus Selector7/1 -> GNSS Receiver Model/4(" Input Voltage (V)")  "<Power Bus: GNSS (signal 4)>"
  Bus Selector6/1 -> Gyroscope Model/2(Input Voltage (V))  "<Power Bus: Gyrospcopes (signal 3)>"
  Transformers1/1 -> Bus Selector3/1
  Bus Selector3/1 -> GNSS Receiver Model/2(ICRF to ITRF TM)  "<ICRF to ITRF TM>"

== system ADCSSimulator/ADCS/ADCS Software/Attitude Control ==
  System Mode : Inport
  Desired Quaternion : Inport  Port=2
  Estimated Attitude State : Inport  Port=3
  Actuators Feedback : Inport  Port=4
  Bus Creator : BusCreator  Inputs=3
  Bus Selector : BusSelector  OutputSignals=Corrected Angular Velocity [Body] (rad/s),Corrected Magnetic Field [Body] (T),Attitude Quaternion [ICRF to Body]
  Bus Selector1 : BusSelector  OutputSignals=Desired Quaternion (Nadir Pointing) [Body to ICRF],Desired Quaternion (Sun Pointing) [ICRF to Body]
  Chart : Stateflow chart  TreatAsAtomicUnit=on
      settings: PortSchema="{\"entries\":[{\"content\":{\"sides\":[{\"content\":{\"connectorIds\":[\"In1\",\"In3\",\"In2\",\"In4\",\"In5\",\"In6\",\"In7\"]},\"type\":\"ConnectorPlacement.EquallySpacedRectSide\",\"uuid\":\"062a988a-98a1-4ae8-a097-d879740615a4\"},{\"content\":{\"connectorIds\":[\"Out1\",\"Out2\",\"Out3\"],\"side\":\"RIGHT\"},\"type\":\"ConnectorPlacement.EquallySpacedRectSide\",\"uuid\":\"dc615fa6-954a-47e4-a374-d574bb9d54f7\"},{\"content\":{\"side\":\"TOP\"},\"type\":\"ConnectorPlacement.EquallySpacedRectSide\",\"uuid\":\"522af153-1f76-4c07-8e9f-67d14e5a0051\"}]},\"type\":\"ConnectorPlacement.EquallySpacedConnector\",\"uuid\":\"61409051-3f1a-4ebe-a56c-175fc221fce9\"}],\"packageUris\":[\"http://schema.mathworks.com/mf0/Connector/R2020b\"],\"version\":\"1.0\"}"
  Wheel Momentum Calculator : Subsystem
  Control Command : Outport
  wires:
  Chart/1(TorqueCommand) -> Bus Creator/1  "Torque Command"
  Chart/2(DipoleCommand) -> Bus Creator/2  "Dipole Command (Given from Torque)"
  Bus Creator/1 -> Control Command/1
  System Mode/1 -> Chart/1(SysMode)
  Estimated Attitude State/1 -> Bus Selector/1
  Bus Selector/1 -> Chart/3(MeasuredAngularVelocity_Body)  "<Corrected Angular Velocity [Body] (rad/s)>"
  Desired Quaternion/1 -> Bus Selector1/1
  Bus Selector/2 -> Chart/2(MeasuredMagneticField_Body)  "<Corrected Magnetic Field [Body] (T)>"
  Bus Selector/3 -> Chart/4(ICRF2BodyQuaternions)  "<Attitude Quaternion [ICRF to Body]>"
  Bus Selector1/1 -> Chart/5(qDesired_NadirPointing)  "<Desired Quaternion (Nadir Pointing) [Body to ICRF]>"
  Bus Selector1/2 -> Chart/6(qDesired_SunPointing)  "<Desired Quaternion (Sun Pointing) [ICRF to Body]>"
  Chart/3(ErrorQuaternion) -> Bus Creator/3  "Error Quaternion [for Pointing Modes]"
  Wheel Momentum Calculator/1(Wheel Momentum Vector) -> Chart/7(Wheel_Momentum_Vector)
  Actuators Feedback/1 -> Wheel Momentum Calculator/1(Actuators Feedback)

== system ADCSSimulator/ADCS/ADCS Software/Attitude Determination ==
  Onboard Models : Inport
  Sensors : Inport  Port=2
  <ICRF to Body Quaternions> : Inport  Port=3
  <ICRF to Body Quaternions>1 : InportShadow  Port=3
  Attitude Estimation Algorithm (MEKF) : Subsystem
  Bus Creator : BusCreator  Inputs=6
  Bus Selector : BusSelector  OutputSignals=Measured Angular Velocity [Body] (rad/s),Measured Magnetic Field [Body] (T)
  Constant : Constant  Value=[0;0;0]
  Onboard Models1 : InportShadow
  Sensors1 : InportShadow  Port=2
  Sensors2 : InportShadow  Port=2
  Static Attitude Determination Algorithm (QUEST) : Subsystem
  Sum : Sum  Inputs=-+|
  Sum1 : Sum  Inputs=-+|
  To Workspace1 : ToWorkspace  VariableName=Quest_lambda  SaveFormat=Timeseries  SampleTime=-1
  Estimated Attitude State : Outport
  wires:
  Onboard Models/1 -> Static Attitude Determination Algorithm (QUEST)/2(Onboard Models)
  Static Attitude Determination Algorithm (QUEST)/3(QUEST: ICRF to Body Quaternion) -> Bus Creator/1, [Quest_Quaternion]  "Static Determination (QUEST): ICRF to Body Quaternion"
  Sensors/1 -> Static Attitude Determination Algorithm (QUEST)/1(Sensors Data)
  Static Attitude Determination Algorithm (QUEST)/1(QUEST: Covariance Matrix) -> [Quest_P]  "Static Determination: Approximated Covariance Matrix"
  Static Attitude Determination Algorithm (QUEST)/2(QUEST: lambda_max) -> [Quest_lambdaMax], To Workspace1/1  "Static Determination: Lambda_max"
  Bus Creator/1 -> Estimated Attitude State/1
  Onboard Models1/1 -> Attitude Estimation Algorithm (MEKF)/2(Onboard Models)
  Sensors1/1 -> Attitude Estimation Algorithm (MEKF)/1(Sensors)
  [Quest_Quaternion] -> Attitude Estimation Algorithm (MEKF)/3(QUEST Quaternion [ICRF to Body])
  <ICRF to Body Quaternions>/1 -> Bus Creator/4  "Attitude Quaternion [ICRF to Body]"
  Attitude Estimation Algorithm (MEKF)/2(State Covariance) -> Bus Creator/3  "State Covariance Matrix"
  Sensors2/1 -> Bus Selector/1
  Bus Selector/1 -> Sum/2  "<Measured Angular Velocity [Body] (rad/s)>"
  Bus Selector/2 -> Sum1/2  "<Measured Magnetic Field [Body] (T)>"
  Sum/1 -> Bus Creator/5  "Corrected Angular Velocity [Body] (rad/s)"
  Sum1/1 -> Bus Creator/6  "Corrected Magnetic Field [Body] (T)"
  Constant/1 -> Sum/1, Sum1/1
  Attitude Estimation Algorithm (MEKF)/1(Attitude Quaternion [ICRF to Body]) -> Bus Creator/2  "Attitude  [ICRF to Body]"
  <ICRF to Body Quaternions>1/1 -> Attitude Estimation Algorithm (MEKF)/4(q_real)  "Attitude Quaternion [ICRF to Body]"

== system ADCSSimulator/ADCS/ADCS Software/Attitude Guidance ==
  Refernce Vectors : Inport
  Transformers : Inport  Port=2
  Bus Creator : BusCreator  Inputs=2
  Bus Selector : BusSelector  OutputSignals=Onboard Sun Ephemeris.Onboard Sun Position [ICRF] (m)
  Bus Selector1 : BusSelector  OutputSignals=Quaternions.ICRF to Orbit Quaternions
  Desired Body to Orbit quaternion [Nadir Pointing] : Constant  Value=[1 ;0 ;0 ;0]
  MATLAB Function : MATLAB Function  TreatAsAtomicUnit=on
  Normalizer5 : Subsystem
  Quaternion Inverse : aerolibutil/Quaternion Inverse
  Quaternion Inverse1 : aerolibutil/Quaternion Inverse
  Quaternion Multiplication : aerolibutil/Quaternion Multiplication
  Sun‐Pointing Body Axis (-Z) : Constant  Value=[0 ;0 ;-1]
  Desired Quaternions : Outport
  wires:
  Refernce Vectors/1 -> Bus Selector/1
  Normalizer5/1(Normalized(A)) -> MATLAB Function/1(sI)  "Sun Position Unit Vector [ICRF]"
  Sun‐Pointing Body Axis (-Z)/1 -> MATLAB Function/2(b_axis)
  MATLAB Function/1(Sun_BodytoICRFQuaternions) -> Bus Creator/1  "Desired Quaternion (Sun Pointing) [ICRF to Body]"
  Bus Selector/1 -> Normalizer5/1(A)  "<Onboard Sun Position [ICRF] (m)>"
  Transformers/1 -> Bus Selector1/1
  Bus Selector1/1 -> Quaternion Multiplication/2  "<ICRF to Orbit Quaternions>"
  Desired Body to Orbit quaternion [Nadir Pointing]/1 -> Quaternion Inverse/1  "Desired Quaternions [Body to Orbit]"
  Quaternion Inverse/1 -> Quaternion Multiplication/1  "Desired Quaternions [Orbit to Body]"
  Bus Creator/1 -> Desired Quaternions/1
  Quaternion Multiplication/1 -> Quaternion Inverse1/1  "Desired Quaternion (Nadir Pointing) [ICRF to Body]"
  Quaternion Inverse1/1 -> Bus Creator/2  "Desired Quaternion (Nadir Pointing) [Body to ICRF]"

== system ADCSSimulator/ADCS/ADCS Software/Normalizer1 ==
  A : Inport
  Dot Product : DotProduct  OutDataTypeStr=Inherit: Inherit via internal rule
  Sqrt1 : Sqrt
  Norm(A) : Outport
  wires:
  Sqrt1/1 -> Norm(A)/1
  A/1 -> Dot Product/2, Dot Product/1
  Dot Product/1 -> Sqrt1/1

== system ADCSSimulator/ADCS/ADCS Software/Normalizer2 ==
  A : Inport
  Dot Product : DotProduct  OutDataTypeStr=Inherit: Inherit via internal rule
  Sqrt1 : Sqrt
  Norm(A) : Outport
  wires:
  Dot Product/1 -> Sqrt1/1
  A/1 -> Dot Product/1, Dot Product/2
  Sqrt1/1 -> Norm(A)/1

== system ADCSSimulator/ADCS/ADCS Software/Normalizer3 ==
  A : Inport
  Dot Product : DotProduct  OutDataTypeStr=Inherit: Inherit via internal rule
  Sqrt1 : Sqrt
  Norm(A) : Outport
  wires:
  Sqrt1/1 -> Norm(A)/1
  A/1 -> Dot Product/2, Dot Product/1
  Dot Product/1 -> Sqrt1/1

== system ADCSSimulator/ADCS/ADCS Software/Normalizer4 ==
  A : Inport
  Dot Product : DotProduct  OutDataTypeStr=Inherit: Inherit via internal rule
  Sqrt1 : Sqrt
  Norm(A) : Outport
  wires:
  Dot Product/1 -> Sqrt1/1
  A/1 -> Dot Product/1, Dot Product/2
  Sqrt1/1 -> Norm(A)/1

== system ADCSSimulator/ADCS/ADCS Software/Normalizer8 ==
  A : Inport
  Dot Product : DotProduct  OutDataTypeStr=Inherit: Inherit via internal rule
  Sqrt1 : Sqrt
  Norm(A) : Outport
  wires:
  Dot Product/1 -> Sqrt1/1
  A/1 -> Dot Product/1, Dot Product/2
  Sqrt1/1 -> Norm(A)/1

== system ADCSSimulator/ADCS/ADCS Software/Onboard Calendar ==
  Calendar Update : Inport
  Bus Selector : BusSelector  Commented=on  OutputSignals=Julian Date (day),Validity Flag
  Calendar Bus Creator : BusCreator  Inputs=4
  Calendar Bus Creator1 : BusCreator  Commented=on  Inputs=4
  Clock Synchronizer : MATLAB Function  Commented=on  TreatAsAtomicUnit=on
  Constant : Constant  Commented=on  Value=2400000.5
  Constant6 : Constant  Value=epoch.DecimalYear
  JD : Subsystem
  JD to Decimal Year : MATLAB Function  Commented=on  TreatAsAtomicUnit=on
  MJD : Subsystem
  "Since Epoch (sec) " : Clock
  Subtract : Sum  Commented=on  Inputs=+-
  Time Step Calculator : Subsystem  Commented=on
  Unit Delay1 : UnitDelay  Commented=on  InitialCondition=2460676.5  SampleTime=-1  HasFrameUpgradeWarning=on
  Calendar : Outport
  wires:
  "Since Epoch (sec) "/1 -> MJD/1(Since Epoch (sec)), JD/1(Since Epoch (sec)), Calendar Bus Creator/4  "Since Epoch (sec)"
  Constant6/1 -> Calendar Bus Creator/3  "Decimal Year (year)"
  JD/1(Julian Date (day)) -> Calendar Bus Creator/1  "Julian Date (day)"
  Calendar Bus Creator/1 -> Calendar/1  "Calendar_out"
  MJD/1(Modified Julian Date (day)) -> Calendar Bus Creator/2  "Modified Julian Date (day)"
  Unit Delay1/1 -> Clock Synchronizer/1(onboard_rtc_julian_date)
  Clock Synchronizer/1(corrected_julian_date_utc) -> JD to Decimal Year/1(jd), Subtract/1, Unit Delay1/1, Calendar Bus Creator1/1  "Julian Date (day)"
  Constant/1 -> Subtract/2
  Subtract/1 -> Calendar Bus Creator1/2  "Modified Julian Date (day)"
  Clock Synchronizer/2(drift_correction_sec) -> Calendar Bus Creator1/4  "RTC Drift"
  JD to Decimal Year/1(dec_year) -> Calendar Bus Creator1/3  "Decimal Year (year)"
  Time Step Calculator/1(dt) -> Clock Synchronizer/4(dt)
  Calendar Update/1 -> Bus Selector/1  "GPS Date"
  Bus Selector/1 -> Clock Synchronizer/2(gps_julian_date)  "<Julian Date (day)>"
  Bus Selector/2 -> Clock Synchronizer/3(is_gps_time_valid)  "<Validity Flag>"
